simulink model "modelVerification"  (R2025a)
settings: Solver=FixedStepDiscrete  StartTime=0.0  StopTime=stopTime  FixedStep=MST  RelTol=1e-3  EnableMultiTasking=on
values from neighbouring files (symbols this model uses):
  lvdtOffsetDig = uint16(adc_kl25z(V_bias))    [verification.m]
  maxRatio = 0.5    [parameters.m]
  maxStroke = 5    [parameters.m]
  samplePeriod = 1/sampleFrequency    (= 0.001)    [parameters.m]
  samplesPerCycle = 332    [parameters.m]
libraries: dspstat3 x6, simulink x2
settings Model: Creator=mbrun  LastModifiedBy=mbrun
settings SFSimCC: MATLABDynamicMemAlloc=off

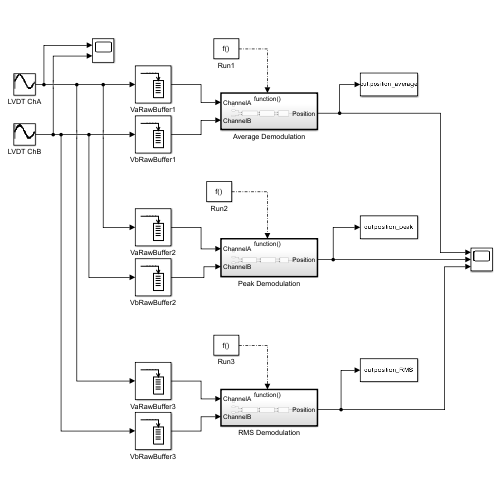
[thumbnail: Simulink's stored preview of the top-level diagram]
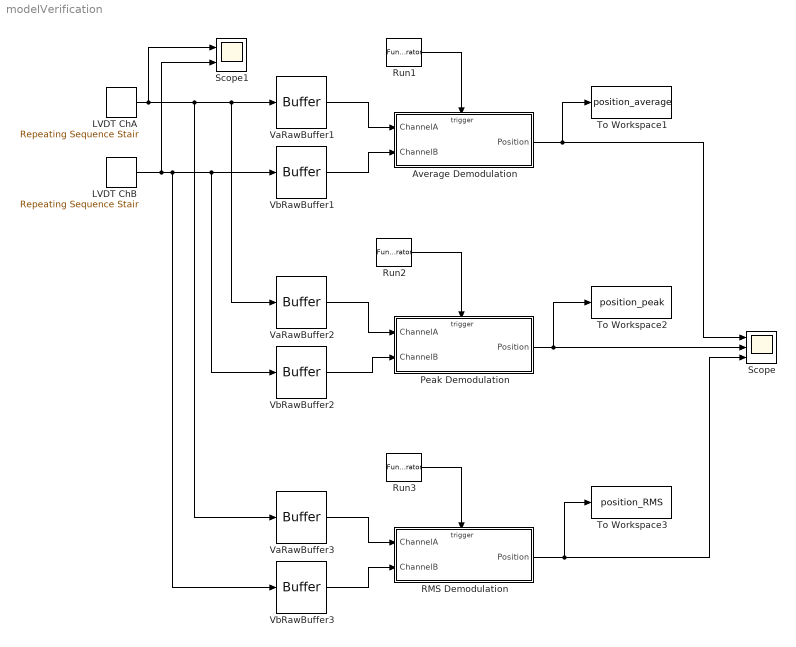
== system modelVerification ==
  Average Demodulation : Subsystem  TreatAsAtomicUnit=on
  LVDT ChA : simulink/Sources/Repeating Sequence Stair  OutValues=adcSignalA  tsamp=samplePeriod  OutMin=[]  OutMax=[]  OutDataTypeStr=uint16  OutputDataTypeScalingMode=uint16  OutDataType=fixdt(0,8)  ConRadixGroup=Best Precision: Vector-wise  OutScaling=2^-12
  LVDT ChB : simulink/Sources/Repeating Sequence Stair  OutValues=adcSignalB  tsamp=samplePeriod  OutMin=[]  OutMax=[]  OutDataTypeStr=uint16  OutputDataTypeScalingMode=uint16  OutDataType=fixdt(0,8)  ConRadixGroup=Best Precision: Vector-wise  OutScaling=2^-12
  Peak Demodulation : Subsystem  TreatAsAtomicUnit=on
  RMS Demodulation : Subsystem  TreatAsAtomicUnit=on
  Run1 : FunctionCallGenerator  SampleTime=samplePeriod*samplesPerCycle
  Run2 : FunctionCallGenerator  SampleTime=samplePeriod*samplesPerCycle
  Run3 : FunctionCallGenerator  SampleTime=samplePeriod*samplesPerCycle
  Scope : Scope  NumInputPorts=3
      settings: ActiveDisplayYMinimum=-11.323972382990879  ActiveDisplayYMaximum=1.9157514469179251
  Scope1 : Scope  NumInputPorts=2
      settings: ActiveDisplayYMinimum=1219.6292603326615  ActiveDisplayYMaximum=2912.129260332661
  To Workspace1 : ToWorkspace  VariableName=position_average  SampleTime=-1
      settings: Save2DSignal=2-D array (concatenate along first dimension)
  To Workspace2 : ToWorkspace  VariableName=position_peak  SampleTime=-1
      settings: Save2DSignal=2-D array (concatenate along first dimension)
  To Workspace3 : ToWorkspace  VariableName=position_RMS  SampleTime=-1
      settings: Save2DSignal=2-D array (concatenate along first dimension)
  VaRawBuffer1 : Buffer  N=samplesPerCycle
  VaRawBuffer2 : Buffer  N=samplesPerCycle
  VaRawBuffer3 : Buffer  N=samplesPerCycle
  VbRawBuffer1 : Buffer  N=samplesPerCycle
  VbRawBuffer2 : Buffer  N=samplesPerCycle
  VbRawBuffer3 : Buffer  N=samplesPerCycle
  wires:
  LVDT ChA/1 -> Scope1/1, VaRawBuffer3/1, VaRawBuffer2/1, VaRawBuffer1/1
  LVDT ChB/1 -> Scope1/2, VbRawBuffer3/1, VbRawBuffer2/1, VbRawBuffer1/1
  Average Demodulation/1(Position) -> Scope/1, To Workspace1/1
  Run1/1 -> Average Demodulation/Trigger
  VbRawBuffer1/1 -> Average Demodulation/2(ChannelB)
  VaRawBuffer1/1 -> Average Demodulation/1(ChannelA)
  Run2/1 -> Peak Demodulation/Trigger
  VaRawBuffer2/1 -> Peak Demodulation/1(ChannelA)
  VbRawBuffer2/1 -> Peak Demodulation/2(ChannelB)
  Peak Demodulation/1(Position) -> To Workspace2/1, Scope/2
  Run3/1 -> RMS Demodulation/Trigger
  VbRawBuffer3/1 -> RMS Demodulation/2(ChannelB)
  VaRawBuffer3/1 -> RMS Demodulation/1(ChannelA)
  RMS Demodulation/1(Position) -> To Workspace3/1, Scope/3

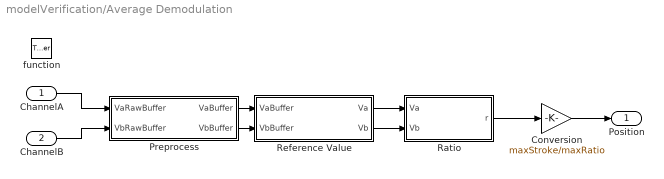
== system modelVerification/Average Demodulation ==
  ChannelA : Inport
  ChannelB : Inport  Port=2
  function : TriggerPort  TriggerType=function-call  VariantControl=(inherit)
  Conversion : Gain  Gain=maxStroke/maxRatio  OutDataTypeStr=double
  Preprocess : Subsystem
  Ratio : Subsystem
  Reference Value : Subsystem
  Position : Outport  OutDataTypeStr=double
  wires:
  Preprocess/2(VbBuffer) -> Reference Value/2(VbBuffer)
  Ratio/1(r) -> Conversion/1
  ChannelB/1 -> Preprocess/2(VbRawBuffer)
  Reference Value/1(Va) -> Ratio/1(Va)
  Preprocess/1(VaBuffer) -> Reference Value/1(VaBuffer)
  Conversion/1 -> Position/1
  Reference Value/2(Vb) -> Ratio/2(Vb)
  ChannelA/1 -> Preprocess/1(VaRawBuffer)

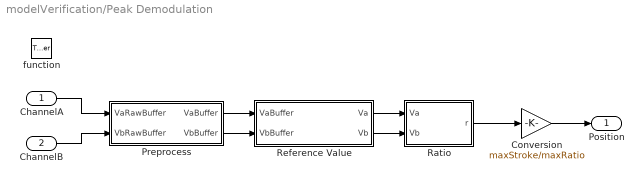
== system modelVerification/Peak Demodulation ==
  ChannelA : Inport
  ChannelB : Inport  Port=2
  function : TriggerPort  TriggerType=function-call  VariantControl=(inherit)
  Conversion : Gain  Gain=maxStroke/maxRatio  OutDataTypeStr=double
  Preprocess : Subsystem
  Ratio : Subsystem
  Reference Value : Subsystem
  Position : Outport  OutDataTypeStr=double
  wires:
  ChannelA/1 -> Preprocess/1(VaRawBuffer)
  Conversion/1 -> Position/1
  Preprocess/2(VbBuffer) -> Reference Value/2(VbBuffer)
  Reference Value/1(Va) -> Ratio/1(Va)
  Preprocess/1(VaBuffer) -> Reference Value/1(VaBuffer)
  Ratio/1(r) -> Conversion/1
  ChannelB/1 -> Preprocess/2(VbRawBuffer)
  Reference Value/2(Vb) -> Ratio/2(Vb)

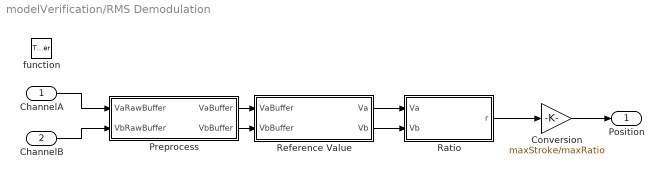
== system modelVerification/RMS Demodulation ==
  ChannelA : Inport
  ChannelB : Inport  Port=2
  function : TriggerPort  TriggerType=function-call  VariantControl=(inherit)
  Conversion : Gain  Gain=maxStroke/maxRatio  OutDataTypeStr=double
  Preprocess : Subsystem
  Ratio : Subsystem
  Reference Value : Subsystem
  Position : Outport  OutDataTypeStr=double
  wires:
  Preprocess/2(VbBuffer) -> Reference Value/2(VbBuffer)
  Ratio/1(r) -> Conversion/1
  ChannelB/1 -> Preprocess/2(VbRawBuffer)
  Reference Value/1(Va) -> Ratio/1(Va)
  Preprocess/1(VaBuffer) -> Reference Value/1(VaBuffer)
  Conversion/1 -> Position/1
  Reference Value/2(Vb) -> Ratio/2(Vb)
  ChannelA/1 -> Preprocess/1(VaRawBuffer)

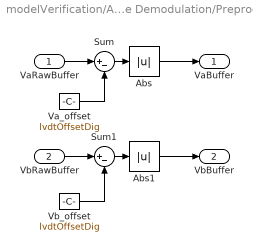
== system modelVerification/Average Demodulation/Preprocess ==
  VaRawBuffer : Inport  OutDataTypeStr=uint16
  VbRawBuffer : Inport  Port=2  OutDataTypeStr=uint16
  Abs : Abs  OutDataTypeStr=double  SaturateOnIntegerOverflow=off
  Abs1 : Abs  OutDataTypeStr=double  SaturateOnIntegerOverflow=off
  Sum : Sum  Inputs=|+-  OutDataTypeStr=double
  Sum1 : Sum  Inputs=|+-  OutDataTypeStr=double
  Va_offset : Constant  Value=lvdtOffsetDig
  Vb_offset : Constant  Value=lvdtOffsetDig
  VaBuffer : Outport  OutDataTypeStr=double
  VbBuffer : Outport  Port=2  OutDataTypeStr=double
  wires:
  Abs/1 -> VaBuffer/1
  Abs1/1 -> VbBuffer/1
  Vb_offset/1 -> Sum1/2
  VaRawBuffer/1 -> Sum/1
  Sum/1 -> Abs/1
  Va_offset/1 -> Sum/2
  Sum1/1 -> Abs1/1
  VbRawBuffer/1 -> Sum1/1

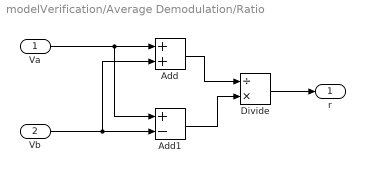
== system modelVerification/Average Demodulation/Ratio ==
  Va : Inport  OutDataTypeStr=double
  Vb : Inport  Port=2  OutDataTypeStr=double
  Add : Sum
  Add1 : Sum  Inputs=+-
  Divide : Product  Inputs=/*
  r : Outport  OutDataTypeStr=double
  wires:
  Vb/1 -> Add/2, Add1/2
  Add1/1 -> Divide/2
  Add/1 -> Divide/1
  Va/1 -> Add1/1, Add/1
  Divide/1 -> r/1

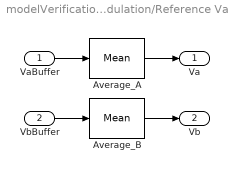
== system modelVerification/Average Demodulation/Reference Value ==
  VaBuffer : Inport  OutDataTypeStr=double
  VbBuffer : Inport  Port=2  OutDataTypeStr=double
  Average_A : dspstat3/Mean  run=off  InputProcessing=Columns as channels (frame based)  reset_popup=None  directionMode=Each column  dimension=1  roiEnable=off  roiType=Rectangles  roiPortion=Entire ROI  roiOutput=Individual statistics for each ROI  roiFlag=off  roundingMode=Floor  overflowMode=off  outputDataTypeStr=Inherit: Same as accumulator  outputMin=[]  outputMax=[]  outputLastDataTypeStr=Inherit: Same as accumulator
  Average_B : dspstat3/Mean  run=off  InputProcessing=Columns as channels (frame based)  reset_popup=None  directionMode=Each column  dimension=1  roiEnable=off  roiType=Rectangles  roiPortion=Entire ROI  roiOutput=Individual statistics for each ROI  roiFlag=off  roundingMode=Floor  overflowMode=off  outputDataTypeStr=Inherit: Same as accumulator  outputMin=[]  outputMax=[]  outputLastDataTypeStr=Inherit: Same as accumulator
  Va : Outport  OutDataTypeStr=double
  Vb : Outport  Port=2  OutDataTypeStr=double
  wires:
  Average_B/1 -> Vb/1
  VaBuffer/1 -> Average_A/1
  Average_A/1 -> Va/1
  VbBuffer/1 -> Average_B/1

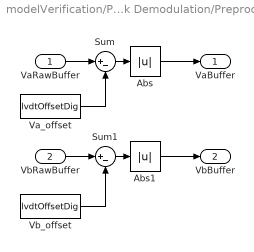
== system modelVerification/Peak Demodulation/Preprocess ==
  VaRawBuffer : Inport  OutDataTypeStr=uint16
  VbRawBuffer : Inport  Port=2  OutDataTypeStr=uint16
  Abs : Abs  OutDataTypeStr=double  SaturateOnIntegerOverflow=off
  Abs1 : Abs  OutDataTypeStr=double  SaturateOnIntegerOverflow=off
  Sum : Sum  Inputs=|+-  OutDataTypeStr=double
  Sum1 : Sum  Inputs=|+-  OutDataTypeStr=double
  Va_offset : Constant  Value=lvdtOffsetDig
  Vb_offset : Constant  Value=lvdtOffsetDig
  VaBuffer : Outport  OutDataTypeStr=double
  VbBuffer : Outport  Port=2  OutDataTypeStr=double
  wires:
  Abs/1 -> VaBuffer/1
  Abs1/1 -> VbBuffer/1
  Vb_offset/1 -> Sum1/2
  VaRawBuffer/1 -> Sum/1
  Sum/1 -> Abs/1
  Va_offset/1 -> Sum/2
  Sum1/1 -> Abs1/1
  VbRawBuffer/1 -> Sum1/1

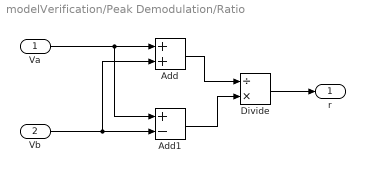
== system modelVerification/Peak Demodulation/Ratio ==
  Va : Inport  OutDataTypeStr=double
  Vb : Inport  Port=2  OutDataTypeStr=double
  Add : Sum
  Add1 : Sum  Inputs=+-
  Divide : Product  Inputs=/*
  r : Outport  OutDataTypeStr=double
  wires:
  Vb/1 -> Add/2, Add1/2
  Add1/1 -> Divide/2
  Add/1 -> Divide/1
  Va/1 -> Add1/1, Add/1
  Divide/1 -> r/1

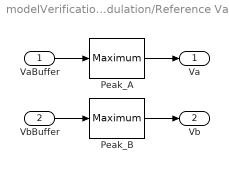
== system modelVerification/Peak Demodulation/Reference Value ==
  VaBuffer : Inport  OutDataTypeStr=double
  VbBuffer : Inport  Port=2  OutDataTypeStr=double
  Peak_A : dspstat3/Maximum  operation=maximum  fcn=Value  indexBase=One  operateOver=Each column  Dimension=1  InputProcessing=Columns as channels (frame based)  reset=None  roiEnable=off  roiType=Rectangles  roiPortion=Entire ROI  roiOutput=Individual statistics for each ROI  roiFlag=off  roundingMode=Floor  overflowMode=off  accumDataTypeStr=Inherit: Same as product output  accumLastDataTypeStr=Inherit: Same as product output
  Peak_B : dspstat3/Maximum  operation=maximum  fcn=Value  indexBase=One  operateOver=Each column  Dimension=1  InputProcessing=Columns as channels (frame based)  reset=None  roiEnable=off  roiType=Rectangles  roiPortion=Entire ROI  roiOutput=Individual statistics for each ROI  roiFlag=off  roundingMode=Floor  overflowMode=off  accumDataTypeStr=Inherit: Same as product output  accumLastDataTypeStr=Inherit: Same as product output
  Va : Outport  OutDataTypeStr=double
  Vb : Outport  Port=2  OutDataTypeStr=double
  wires:
  Peak_B/1 -> Vb/1
  VaBuffer/1 -> Peak_A/1
  VbBuffer/1 -> Peak_B/1
  Peak_A/1 -> Va/1

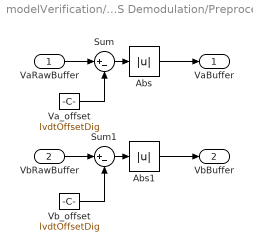
== system modelVerification/RMS Demodulation/Preprocess ==
  VaRawBuffer : Inport  OutDataTypeStr=uint16
  VbRawBuffer : Inport  Port=2  OutDataTypeStr=uint16
  Abs : Abs  OutDataTypeStr=double  SaturateOnIntegerOverflow=off
  Abs1 : Abs  OutDataTypeStr=double  SaturateOnIntegerOverflow=off
  Sum : Sum  Inputs=|+-  OutDataTypeStr=double
  Sum1 : Sum  Inputs=|+-  OutDataTypeStr=double
  Va_offset : Constant  Value=lvdtOffsetDig
  Vb_offset : Constant  Value=lvdtOffsetDig
  VaBuffer : Outport  OutDataTypeStr=double
  VbBuffer : Outport  Port=2  OutDataTypeStr=double
  wires:
  Abs/1 -> VaBuffer/1
  Abs1/1 -> VbBuffer/1
  Vb_offset/1 -> Sum1/2
  VaRawBuffer/1 -> Sum/1
  Sum/1 -> Abs/1
  Va_offset/1 -> Sum/2
  Sum1/1 -> Abs1/1
  VbRawBuffer/1 -> Sum1/1

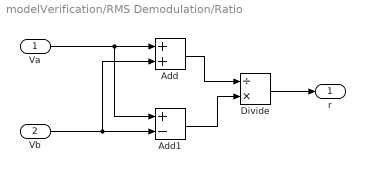
== system modelVerification/RMS Demodulation/Ratio ==
  Va : Inport  OutDataTypeStr=double
  Vb : Inport  Port=2  OutDataTypeStr=double
  Add : Sum
  Add1 : Sum  Inputs=+-
  Divide : Product  Inputs=/*
  r : Outport  OutDataTypeStr=double
  wires:
  Vb/1 -> Add/2, Add1/2
  Add1/1 -> Divide/2
  Add/1 -> Divide/1
  Va/1 -> Add1/1, Add/1
  Divide/1 -> r/1

== system modelVerification/RMS Demodulation/Reference Value ==
  VaBuffer : Inport  OutDataTypeStr=double
  VbBuffer : Inport  Port=2  OutDataTypeStr=double
  RMS_A : dspstat3/RMS  run=off  directionMode=Each column  dimension=1  InputProcessing=Columns as channels (frame based)  reset_popup=None
  RMS_B : dspstat3/RMS  run=off  directionMode=Each column  dimension=1  InputProcessing=Columns as channels (frame based)  reset_popup=None
  Va : Outport  OutDataTypeStr=double
  Vb : Outport  Port=2  OutDataTypeStr=double
  wires:
  VaBuffer/1 -> RMS_A/1
  RMS_A/1 -> Va/1
  VbBuffer/1 -> RMS_B/1
  RMS_B/1 -> Vb/1
